simulink subsystem "max_margin_controller"  (R2024b)
settings: Solver=VariableStepAuto  StartTime=0.0  StopTime=10.0  RelTol=1e-3
undefined symbols (not defined in the file): const_brake, controller_rate, Kp, target_const_effort
libraries: simulink x1
settings Model: Creator=yevge  LastModifiedBy=Aiden Gaydos

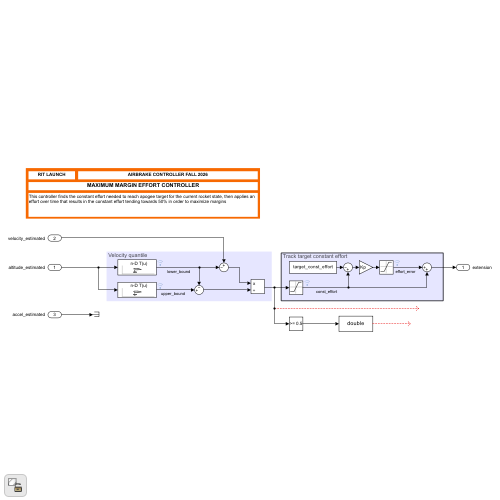
[thumbnail: Simulink's stored preview of the top-level diagram]
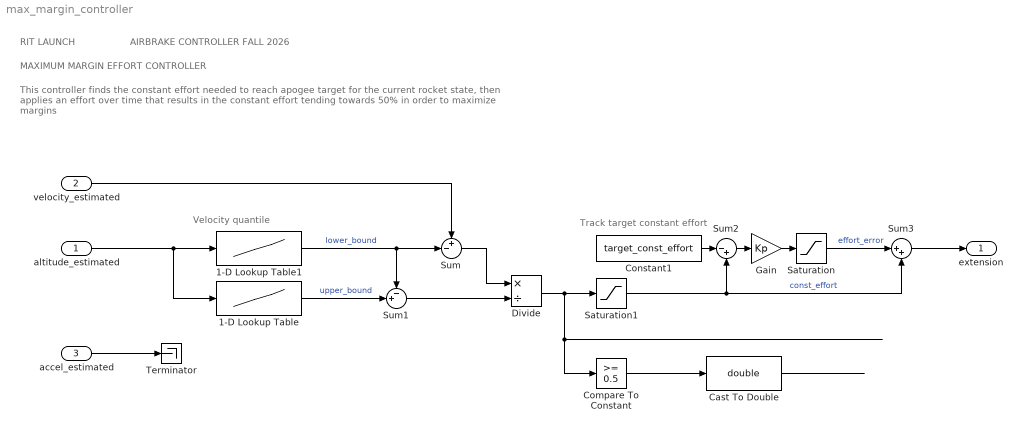
== system max_margin_controller ==
  note: Track target constant effort
  note: Velocity quantile
  note: MAXIMUM MARGIN EFFORT CONTROLLER
  note: This controller finds the constant effort needed to reach apogee target for the current rocket state, then applies an effort over time that results in the constant effort tending towards 50% in order to maximize margins
  note: RIT LAUNCH
  note: AIRBRAKE CONTROLLER FALL 2026
  altitude_estimated : Inport  Unit=m  PortDimensions=1
  velocity_estimated : Inport  Port=2  Unit=m/s  PortDimensions=1
  accel_estimated : Inport  Port=3  Unit=m/s^2  PortDimensions=1
  1-D Lookup Table : Lookup_n-D  NumberOfTableDimensions=1  DataSpecification=Lookup table object  LookupTableObject=upper_bound_lut  BreakpointsForDimension1=[-5:5]  Table=tanh([-5:5])  InternalRulePriority=Speed  RndMeth=Simplest
  1-D Lookup Table1 : Lookup_n-D  NumberOfTableDimensions=1  DataSpecification=Lookup table object  LookupTableObject=lower_bound_lut  BreakpointsForDimension1=[-5:5]  Table=tanh([-5:5])  InternalRulePriority=Speed  RndMeth=Simplest
  Cast To Double : DataTypeConversion  OutDataTypeStr=double  SaturateOnIntegerOverflow=off  RndMeth=Floor
  Compare To Constant : simulink/Logic and Bit Operations/Compare To Constant  relop=>=  const=0.5  OutDataTypeStr=boolean
  Constant1 : Constant  Value=target_const_effort
  Divide : Product  Inputs=*/
  Gain : Gain  Gain=Kp
  Saturation : Saturate  UpperLimit=1  LowerLimit=-1
  Saturation1 : Saturate  UpperLimit=1  LowerLimit=0
  Sum : Sum  Inputs=+-|
  Sum1 : Sum  Inputs=-+|
  Sum2 : Sum  Inputs=|-+
  Sum3 : Sum  Inputs=|++
  Terminator : Terminator
  extension : Outport  Unit=1  PortDimensions=1  SampleTime=1/controller_rate  InitialOutput=const_brake
  wires:
  accel_estimated/1 -> Terminator/1
  altitude_estimated/1 -> 1-D Lookup Table/1, 1-D Lookup Table1/1
  1-D Lookup Table1/1 -> Sum1/1, Sum/2  "lower_bound"
  1-D Lookup Table/1 -> Sum1/2  "upper_bound"
  Sum/1 -> Divide/1
  Sum1/1 -> Divide/2
  velocity_estimated/1 -> Sum/1
  Sum2/1 -> Gain/1
  Sum3/1 -> extension/1
  Divide/1 -> Saturation1/1, Compare To Constant/1
  Saturation/1 -> Sum3/1  "effort_error"
  Saturation1/1 -> Sum2/2, Sum3/2  "const_effort"
  Gain/1 -> Saturation/1
  Constant1/1 -> Sum2/1
  Compare To Constant/1 -> Cast To Double/1
  Cast To Double/1 -> ?
